simulink model "R2026b_pv_inverter_L_LC"  (R2026b)
settings: Solver=ode23tb  StopTime=0.3  MaxStep=2e-6  RelTol=1e-4  AbsTol=1e-6
libraries: ee_lib x13, nesl_utility x13, fl_lib x7
settings Model: Creator=35015  LastModifiedBy=35015
settings SimscapeCC: SimscapeLogType=all  SimscapeNominalValues="[{\"value\":\"1\",\"unit\":\"A\"},{\"value\":\"1\",\"unit\":\"bar\"},{\"value\":\"1\",\"unit\":\"cm^2\"},{\"value\":\"1\",\"unit\":\"cm^3/s\"},{\"value\":\"1\",\"unit\":\"kJ/kg\"},{\"value\":\"1\",\"unit\":\"kW\"},{\"value\":\"1\",\"unit\":\"l\"},{\"value\":\"1\",\"unit\":\"N\"},{\"value\":\"1\",\"unit\":\"N*m\"},{\"value\":\"1\",\"unit\":\"V\"},{\"value\":\"0.001\",\"unit\":\"Wb\"}]"  SimscapeUseEnergyAccounting=off

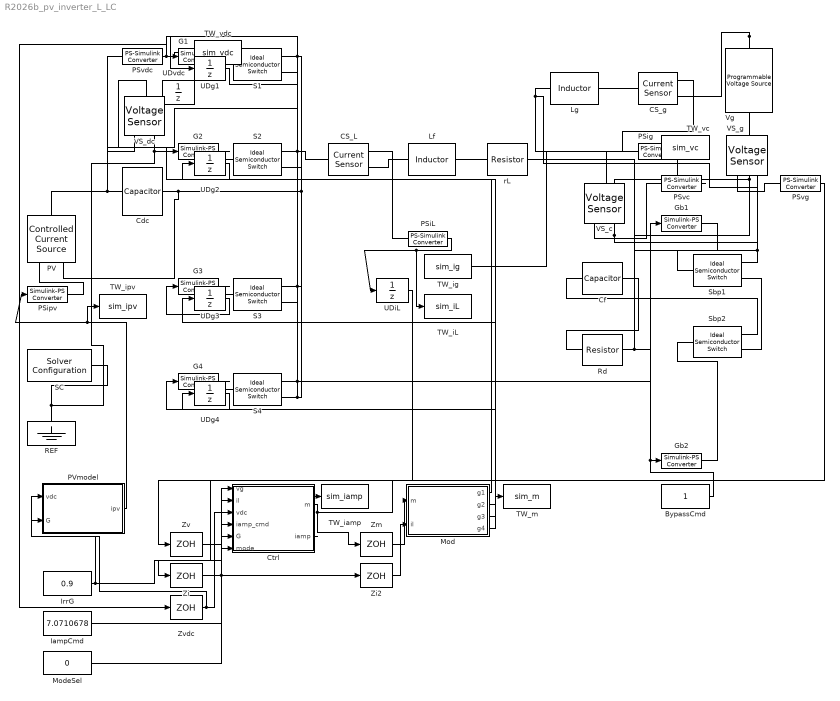
== system R2026b_pv_inverter_L_LC ==
  BypassCmd : Constant
  CS_L : fl_lib/Electrical/Electrical Sensors/Current Sensor
  CS_g : fl_lib/Electrical/Electrical Sensors/Current Sensor
  Cdc : ee_lib/Passive/Capacitor  cap_option=ee.enum.passive.capacitor.capOption.const  c=0.0045 F  Cvec=[1e-05, 1e-06] F  Vvec=[0, 10] V  CV_table_symmetry=ee.enum.passive.capacitor.tableSymmetry.yes  f_vec=[1, 10] kHz  DFext_vec=[.8, 1.2]  enable_C_tol=ee.enum.toleranceApplication.none  averaging_period=0 s  C_tol=5  tol_distribution=ee.enum.toleranceDistribution.uniform  nSigma=4  r=0 Ohm  g=0 1/Ohm  enable_operating_limits=ee.enum.enable.no  operating_limit_action=ee.enum.passive.reportOpLim.warn  max_working_voltage_range=[-25, 25] V  power_rating=1 W  maxTemperature=85 degC  thermalEnable=false  thermalMass=1 J/K  i_specify=off  i_priority=None  i=0 A  i_nominal_specify=off  i_nominal_value=1  i_nominal_unit=A  v_specify=off  v_priority=None  v=0 V  v_nominal_specify=off  v_nominal_value=1  v_nominal_unit=V  vc_specify=on  vc_priority=High  vc=75 V  vc_nominal_specify=off  vc_nominal_value=1  vc_nominal_unit=V  T_specify=off  T_priority=None  T=298.15 K  T_nominal_specify=off  T_nominal_value=1  T_nominal_unit=K
  Cf : ee_lib/Passive/Capacitor  cap_option=ee.enum.passive.capacitor.capOption.const  c=2e-05 F  Cvec=[1e-05, 1e-06] F  Vvec=[0, 10] V  CV_table_symmetry=ee.enum.passive.capacitor.tableSymmetry.yes  f_vec=[1, 10] kHz  DFext_vec=[.8, 1.2]  enable_C_tol=ee.enum.toleranceApplication.none  averaging_period=0 s  C_tol=5  tol_distribution=ee.enum.toleranceDistribution.uniform  nSigma=4  r=0 Ohm  g=0 1/Ohm  enable_operating_limits=ee.enum.enable.no  operating_limit_action=ee.enum.passive.reportOpLim.warn  max_working_voltage_range=[-25, 25] V  power_rating=1 W  maxTemperature=85 degC  thermalEnable=false  thermalMass=1 J/K  i_specify=off  i_priority=None  i=0 A  i_nominal_specify=off  i_nominal_value=1  i_nominal_unit=A  v_specify=off  v_priority=None  v=0 V  v_nominal_specify=off  v_nominal_value=1  v_nominal_unit=V  vc_specify=off  vc_priority=High  vc=0 V  vc_nominal_specify=off  vc_nominal_value=1  vc_nominal_unit=V  T_specify=off  T_priority=None  T=298.15 K  T_nominal_specify=off  T_nominal_value=1  T_nominal_unit=K
  Ctrl : MATLAB Function  TreatAsAtomicUnit=on
  G{1..4} (4 alike) : nesl_utility/Simulink-PS Converter  PhysicalDomain=network_engine_domain  SubClassName=ps_input  LeftPortType=input  RightPortType=output  PseudoPeriodic=off  Frequencies=[]  NoiseDistribution=none  NoiseParameters=[]  Unit=V  AffineConversion=off  FilteringAndDerivatives=provide  SimscapeFilterOrder=1  InputFilterTimeConstant=0.001  UdotUserProvided=0
  Gb1 : nesl_utility/Simulink-PS Converter  PhysicalDomain=network_engine_domain  SubClassName=ps_input  LeftPortType=input  RightPortType=output  PseudoPeriodic=off  Frequencies=[]  NoiseDistribution=none  NoiseParameters=[]  Unit=V  AffineConversion=off  FilteringAndDerivatives=provide  SimscapeFilterOrder=1  InputFilterTimeConstant=0.001  UdotUserProvided=0
  Gb2 : nesl_utility/Simulink-PS Converter  PhysicalDomain=network_engine_domain  SubClassName=ps_input  LeftPortType=input  RightPortType=output  PseudoPeriodic=off  Frequencies=[]  NoiseDistribution=none  NoiseParameters=[]  Unit=V  AffineConversion=off  FilteringAndDerivatives=provide  SimscapeFilterOrder=1  InputFilterTimeConstant=0.001  UdotUserProvided=0
  IampCmd : Constant  Value=7.0710678
  IrrG : Constant  Value=0.9
  Lf : ee_lib/Passive/Inductor  l=0.0005 H  enable_L_tol=ee.enum.toleranceApplication.none  L_tol=20  tol_distribution=ee.enum.toleranceDistribution.uniform  nSigma=4  r=0 Ohm  g=1e-9 1/Ohm  enable_operating_limits=ee.enum.enable.no  operating_limit_action=ee.enum.passive.reportOpLim.warn  max_working_current=1 A  power_rating=1 W  i_L_specify=off  i_L_priority=High  i_L=0 A  i_L_nominal_specify=off  i_L_nominal_value=1  i_L_nominal_unit=A
  Lg : ee_lib/Passive/Inductor  l=0.0005 H  enable_L_tol=ee.enum.toleranceApplication.none  L_tol=20  tol_distribution=ee.enum.toleranceDistribution.uniform  nSigma=4  r=0 Ohm  g=1e-9 1/Ohm  enable_operating_limits=ee.enum.enable.no  operating_limit_action=ee.enum.passive.reportOpLim.warn  max_working_current=1 A  power_rating=1 W  i_L_specify=off  i_L_priority=High  i_L=0 A  i_L_nominal_specify=off  i_L_nominal_value=1  i_L_nominal_unit=A
  Mod : MATLAB Function  TreatAsAtomicUnit=on
  ModeSel : Constant  Value=0
  PSiL : nesl_utility/PS-Simulink Converter  PhysicalDomain=network_engine_domain  SubClassName=ps_output  LeftPortType=input  RightPortType=output  PseudoPeriodic=off  Frequencies=[]  VectorFormat=inherit  Unit=A  AffineConversion=off
  PSig : nesl_utility/PS-Simulink Converter  PhysicalDomain=network_engine_domain  SubClassName=ps_output  LeftPortType=input  RightPortType=output  PseudoPeriodic=off  Frequencies=[]  VectorFormat=inherit  Unit=A  AffineConversion=off
  PSipv : nesl_utility/Simulink-PS Converter  PhysicalDomain=network_engine_domain  SubClassName=ps_input  LeftPortType=input  RightPortType=output  PseudoPeriodic=off  Frequencies=[]  NoiseDistribution=none  NoiseParameters=[]  Unit=A  AffineConversion=off  FilteringAndDerivatives=provide  SimscapeFilterOrder=1  InputFilterTimeConstant=0.001  UdotUserProvided=0
  PSvc : nesl_utility/PS-Simulink Converter  PhysicalDomain=network_engine_domain  SubClassName=ps_output  LeftPortType=input  RightPortType=output  PseudoPeriodic=off  Frequencies=[]  VectorFormat=inherit  Unit=V  AffineConversion=off
  PSvdc : nesl_utility/PS-Simulink Converter  PhysicalDomain=network_engine_domain  SubClassName=ps_output  LeftPortType=input  RightPortType=output  PseudoPeriodic=off  Frequencies=[]  VectorFormat=inherit  Unit=V  AffineConversion=off
  PSvg : nesl_utility/PS-Simulink Converter  PhysicalDomain=network_engine_domain  SubClassName=ps_output  LeftPortType=input  RightPortType=output  PseudoPeriodic=off  Frequencies=[]  VectorFormat=inherit  Unit=V  AffineConversion=off
  PV : fl_lib/Electrical/Electrical Sources/Controlled Current Source
  PVmodel : MATLAB Function  TreatAsAtomicUnit=on
  REF : fl_lib/Electrical/Electrical Elements/Electrical Reference
  Rd : ee_lib/Passive/Resistor  R=0.001 Ohm  enable_R_tol=ee.enum.toleranceApplication.none  R_tol=5  tol_distribution=ee.enum.toleranceDistribution.uniform  nSigma=4  enable_operating_limits=ee.enum.enable.no  operating_limit_action=ee.enum.passive.reportOpLim.warn  power_rating=1 W  max_working_voltage=100 V  noise_mode=ee.enum.sources.noise.Disabled  Tdevice=25 degC  sample_time=1e-3 s  repeatability=ee.enum.ic.repeatability.notRepeatable  user_seed=0  auto_seed=3890346746  power_derating_T1=70 degC  power_derating_T2=155 degC  operating_temperature_range_vec=[-50, 150] degC  alpha=3.93e-3 1/K  Tmeas=25 degC  thermal_mass=100 J/K  temperature_specify=off  temperature_priority=High  temperature=298.15 K  temperature_nominal_specify=off  temperature_nominal_value=1  temperature_nominal_unit=K
  S{1..4} (4 alike) : ee_lib/Semiconductors & Converters/Ideal Semiconductor Switch  port_option=ee.enum.controlport.ps  Ron=0.001 Ohm  Goff=1e-6 1/Ohm  Vth=0.5 V  diode_param=ee.enum.semiconductors.protectionDiode.nodynamics  diode_Vf=0.8 V  diode_Ron=0.001 Ohm  diode_Goff=1e-5 1/Ohm  diode_C=50e-9 F  diode_iRM=-235 A  diode_iF=300 A  diode_idot=-50 A/us  diode_trr_param=ee.enum.converters.diodetrr.trr_factor  diode_trr_factor=3  diode_trr=15 us  diode_Qrr=1500 s*uA
  SC : nesl_utility/Solver Configuration  PhysicalDomain=network_engine_domain  SubClassName=solver  LeftPortType=input  RightPortType=generic  Tones=[]  Harmonics=[]  SimulateNoise=off  Profile=off  UseLocalSampling=off  EnableSwitchedLinearOptims=on  FrequencyDomain=off  UseCCode=off  RelTol=0.001  AbsTol=0.001  MinStep=1e-09  ToWorkspace=off  RevertToSquareIcSolve=off  NumHomotopyIterations=100  PhasorMode=off  PhasorModeNumHarmonics=1  ConsistencySolver=NEWTON_XTOL_AFTER_FTOL  CanonicalOrdering=CANONICAL  OptimizeIntermediates=OPTIMIZED  MulticoreSolverChoice=BACKWARD_EULER  IndexReductionMethod=DerivativeReplacement  DoDC=off  ResidualTolerance=1e-09  ConsistencyTolSource=GLOBAL  ConsistencyAbsTol=0.001  ConsistencyRelTol=0.001  ConsistencyTolFactor=0.001  UseLocalSolver=off  LocalSolverChoice=NE_BACKWARD_EULER_ADVANCER  ResolveIndetEquations=on  FunctionEvalNumThread=1  LocalSolverSampleTime=0.001  DoFixedCost=off  MaxNonlinIter=3  MaxModeIter=2  ComputeImpulses=off  ImpulseIterations=2  LinearAlgebra=auto  LinearAlgebraNumThread=0  EquationFormulation=NE_TIME_EF  DelaysMemoryBudget=1024  AutomaticFiltering=on  FilteringTimeConstant=0.001  PartitionStorageMethod=AS_NEEDED  PartitionMemoryBudget=1024  PartitionMethod=BALANCED  MultibodyUseLocalSolver=off  MultibodyLocalSolverChoice=ODE1  MultibodyLocalSolverSampleTime=0.001
  Sbp1 : ee_lib/Semiconductors & Converters/Ideal Semiconductor Switch  port_option=ee.enum.controlport.ps  Ron=0.001 Ohm  Goff=1e-6 1/Ohm  Vth=0.5 V  diode_param=ee.enum.semiconductors.protectionDiode.nodynamics  diode_Vf=0.8 V  diode_Ron=0.001 Ohm  diode_Goff=1e-5 1/Ohm  diode_C=50e-9 F  diode_iRM=-235 A  diode_iF=300 A  diode_idot=-50 A/us  diode_trr_param=ee.enum.converters.diodetrr.trr_factor  diode_trr_factor=3  diode_trr=15 us  diode_Qrr=1500 s*uA
  Sbp2 : ee_lib/Semiconductors & Converters/Ideal Semiconductor Switch  port_option=ee.enum.controlport.ps  Ron=0.001 Ohm  Goff=1e-6 1/Ohm  Vth=0.5 V  diode_param=ee.enum.semiconductors.protectionDiode.nodynamics  diode_Vf=0.8 V  diode_Ron=0.001 Ohm  diode_Goff=1e-5 1/Ohm  diode_C=50e-9 F  diode_iRM=-235 A  diode_iF=300 A  diode_idot=-50 A/us  diode_trr_param=ee.enum.converters.diodetrr.trr_factor  diode_trr_factor=3  diode_trr=15 us  diode_Qrr=1500 s*uA
  TW_iL : ToWorkspace  VariableName=sim_iL  SaveFormat=Timeseries  SampleTime=2.5e-6
  TW_iamp : ToWorkspace  VariableName=sim_iamp  SaveFormat=Timeseries  SampleTime=5e-5
  TW_ig : ToWorkspace  VariableName=sim_ig  SaveFormat=Timeseries  SampleTime=2.5e-6
  TW_ipv : ToWorkspace  VariableName=sim_ipv  SaveFormat=Timeseries  SampleTime=2.5e-6
  TW_m : ToWorkspace  VariableName=sim_m  SaveFormat=Timeseries  SampleTime=5e-5
  TW_vc : ToWorkspace  VariableName=sim_vc  SaveFormat=Timeseries  SampleTime=2.5e-6
  TW_vdc : ToWorkspace  VariableName=sim_vdc  SaveFormat=Timeseries  SampleTime=2.5e-6
  UDg{1..4} (4 alike) : UnitDelay  SampleTime=2.5e-6
  UDiL : UnitDelay  SampleTime=2.5e-6
  UDvdc : UnitDelay  SampleTime=2.5e-6
  VS_c : fl_lib/Electrical/Electrical Sensors/Voltage Sensor
  VS_dc : fl_lib/Electrical/Electrical Sensors/Voltage Sensor
  VS_g : fl_lib/Electrical/Electrical Sensors/Voltage Sensor
  Vg : ee_lib/Sources/Programmable Voltage Source  magnitude_type=ee.enum.timechanging.constant  ac_magnitude=50.91168825 V  magn_ramp=1 V/s  magn_step=1 V  magn_modu_magn=1 V  magn_modu_freq=1 Hz  magn_t1=1 s  magn_t2=2 s  frequency_type=ee.enum.timechanging.constant  ac_frequency=50 Hz  freq_ramp=1 Hz/s  freq_step=1 Hz  freq_modu_magn=1 Hz  freq_modu_freq=1 Hz  freq_t1=1 s  freq_t2=2 s  phase_type=ee.enum.timechanging.constant  ac_shift=0 deg  phase_ramp=1 deg/s  phase_step=1 deg  phase_modu_magn=1 deg  phase_modu_freq=1 Hz  phase_t1=1 s  phase_t2=2 s  dc_type=ee.enum.timechanging.constant  dc_voltage=0 V  dc_ramp=1 V/s  dc_step=1 V  dc_modu_magn=1 V  dc_modu_freq=1 Hz  dc_t1=1 s  dc_t2=2 s  harmonic_option=0  harmonic_orders=[5, 7, 11, 13]  harmonic_ratios=[.1, .1, .1, .1]  harmonic_shifts=[0, 0, 0, 0] deg  harmonic_t1=-inf s  harmonic_t2=inf s  noise_mode=0  PSD=0 V^2/Hz  repeatability=1  auto_seed=0  user_seed=0  sample_time=1e-3 s  i_specify=off  i_priority=None  i=0 A  i_nominal_specify=off  i_nominal_value=1  i_nominal_unit=A  v_specify=off  v_priority=None  v=0 V  v_nominal_specify=off  v_nominal_value=1  v_nominal_unit=V
  Zi : ZeroOrderHold  SampleTime=5e-5
  Zi2 : ZeroOrderHold  SampleTime=2.5e-6
  Zm : ZeroOrderHold  SampleTime=2.5e-6
  Zv : ZeroOrderHold  SampleTime=5e-5
  Zvdc : ZeroOrderHold  SampleTime=5e-5
  rL : ee_lib/Passive/Resistor  R=0.1 Ohm  enable_R_tol=ee.enum.toleranceApplication.none  R_tol=5  tol_distribution=ee.enum.toleranceDistribution.uniform  nSigma=4  enable_operating_limits=ee.enum.enable.no  operating_limit_action=ee.enum.passive.reportOpLim.warn  power_rating=1 W  max_working_voltage=100 V  noise_mode=ee.enum.sources.noise.Disabled  Tdevice=25 degC  sample_time=1e-3 s  repeatability=ee.enum.ic.repeatability.notRepeatable  user_seed=0  auto_seed=3499211588  power_derating_T1=70 degC  power_derating_T2=155 degC  operating_temperature_range_vec=[-50, 150] degC  alpha=3.93e-3 1/K  Tmeas=25 degC  thermal_mass=100 J/K  temperature_specify=off  temperature_priority=High  temperature=298.15 K  temperature_nominal_specify=off  temperature_nominal_value=1  temperature_nominal_unit=K
  wires:
  PSvdc/1 -> Zvdc/1, TW_vdc/1
  PSvg/1 -> Zv/1
  PSiL/1 -> UDiL/1, TW_iL/1
  UDiL/1 -> Zi/1
  Zvdc/1 -> PVmodel/1(vdc), Ctrl/3(vdc)
  IrrG/1 -> PVmodel/2(G), Ctrl/5(G)
  PVmodel/1(ipv) -> PSipv/1, TW_ipv/1
  Zv/1 -> Ctrl/1(vg)
  Zi/1 -> Ctrl/2(il), Zi2/1
  IampCmd/1 -> Ctrl/4(iamp_cmd)
  ModeSel/1 -> Ctrl/6(mode)
  Ctrl/1(m) -> Zm/1, TW_m/1
  Zm/1 -> Mod/1(m)
  Zi2/1 -> Mod/2(il)
  Mod/1(g1) -> UDg1/1
  Mod/2(g2) -> UDg2/1
  Mod/3(g3) -> UDg3/1
  Mod/4(g4) -> UDg4/1
  UDg1/1 -> G1/1
  UDg2/1 -> G2/1
  UDg3/1 -> G3/1
  UDg4/1 -> G4/1
  BypassCmd/1 -> Gb1/1, Gb2/1
  PSig/1 -> TW_ig/1
  PSvc/1 -> TW_vc/1
  Ctrl/2(iamp) -> TW_iamp/1
  connections:
  PV/LConn1 -- Cdc/LConn1 -- S1/RConn1 -- S3/RConn1 -- VS_dc/LConn1
  PV/RConn2 -- Cdc/RConn1 -- S2/RConn2 -- S4/RConn2 -- VS_dc/RConn2 -- REF/LConn1 -- SC/RConn1
  S1/RConn2 -- S2/RConn1 -- CS_L/LConn1
  CS_L/RConn2 -- Lf/LConn1
  Lf/RConn1 -- rL/LConn1
  rL/RConn1 -- Sbp1/RConn1 -- Lg/LConn1 -- VS_c/LConn1
  Sbp1/RConn2 -- Sbp2/RConn2
  Sbp2/RConn1 -- Cf/LConn1
  Cf/RConn1 -- Rd/LConn1
  S3/RConn2 -- S4/RConn1 -- Rd/RConn1 -- Vg/RConn1 -- VS_c/RConn2 -- VS_g/RConn2
  Lg/RConn1 -- CS_g/LConn1
  Vg/LConn1 -- CS_g/RConn2 -- VS_g/LConn1
  CS_L/RConn1 -- PSiL/LConn1
  CS_g/RConn1 -- PSig/LConn1
  VS_dc/RConn1 -- PSvdc/LConn1
  VS_c/RConn1 -- PSvc/LConn1
  VS_g/RConn1 -- PSvg/LConn1
  PV/RConn1 -- PSipv/RConn1
  G1/RConn1 -- S1/LConn1
  G2/RConn1 -- S2/LConn1
  G3/RConn1 -- S3/LConn1
  G4/RConn1 -- S4/LConn1
  Gb1/RConn1 -- Sbp1/LConn1
  Gb2/RConn1 -- Sbp2/LConn1

== matlab function R2026b_pv_inverter_L_LC/Ctrl ==
  settings: updateMethod=DISCRETE  sampleTime=5e-5
  data: vg input; m output; il input; vdc input; iamp_cmd input; G input; mode input; iamp output
function [m, iamp] = ctrl(vg, il, vdc, iamp_cmd, G, mode)
%#codegen
% SOGI-PLL + 准PR(Tustin预畸变) + 电压环PI + P&O, 与 control_algos.py 同参数
Ts = 5e-5;
persistent th ia ib wq pii y1 y2 e1 e2 vint cnt pacc pn vref lastp dirp iampp init
if isempty(init)
    th = 0; ia = 0; ib = 0; wq = 2*pi*50; pii = 0;
    y1 = 0; y2 = 0; e1 = 0; e2 = 0; vint = 0;
    cnt = 0; pacc = 0; pn = 0; vref = 0.8*90; lastp = -1; dirp = 1; iampp = 0;
    init = 1;
end
w0 = 2*pi*50; ks = 1.41; kpp = 0.67; kip = 22; Um = 36*sqrt(2);
kppr = 4.7; kr = 300; wc = 5;
kpv = 0.2; kiv = 5; imin = 0; imax = 10;
dv = 0.5; vmin = 62; vmax = 75;
fsw = 20000; td = 4e-07; mlim = 0.95;
Iph = 2.9; I0 = 4.05e-8; nVT = 4.95;
kk = w0/tan(w0*Ts/2);
a0 = kk*kk + 2*wc*kk + w0*w0;
b0 = 2*kr*wc*kk/a0;
b2 = -2*kr*wc*kk/a0;
a1 = (-2*kk*kk + 2*w0*w0)/a0;
a2 = (kk*kk - 2*wc*kk + w0*w0)/a0;
% ---- SOGI-PLL ----
ia = ia + Ts*(ks*wq*(vg - ia) - wq*ib);
ib = ib + Ts*(wq*ia);
vq = ia*cos(th) + ib*sin(th);
vqn = vq/Um;
pii = pii + kip*vqn*Ts;
wq = w0 + kpp*vqn + pii;
th = th + wq*Ts;
if th > 2*pi
    th = th - 2*pi;
end
% ---- 电流幅值指令 ----
if mode < 0.5
    iampp = iamp_cmd;
else
    ipv = G*Iph - I0*(exp(vdc/nVT) - 1.0);
    pacc = pacc + vdc*ipv; pn = pn + 1;
    if mod(cnt, 20) == 0
        err = vdc - vref;
        o = kpv*err + vint;
        if ~((o >= imax && err > 0) || (o <= imin && err < 0))
            vint = vint + kiv*err*20*Ts;
        end
        iampp = kpv*err + vint;
        if iampp > imax, iampp = imax; end
        if iampp < imin, iampp = imin; end
    end
    if mod(cnt, 2000) == 0 && pn > 0
        pavg = pacc/pn;
        if lastp >= 0
            if pavg - lastp < 0
                dirp = -dirp;
            end
            vref = vref + dirp*dv;
            if vref > vmax, vref = vmax; end
            if vref < vmin, vref = vmin; end
        end
        lastp = pavg; pacc = 0; pn = 0;
    end
end
iamp = iampp;
% ---- 准PR 电流环 + 电网前馈 + 死区补偿 ----
iref = iamp*sin(th);
e = iref - il;
y = b0*e + b2*e2 - a1*y1 - a2*y2;
e2 = e1; e1 = e; y2 = y1; y1 = y;
u = kppr*e + y + vg;
u = u + 2*fsw*td*vdc*(1 - 2*(il < 0));
vdcs = vdc;
if vdcs < 10, vdcs = 10; end
lim = mlim*vdcs;
if u > lim, u = lim; end
if u < -lim, u = -lim; end
m = u/vdcs;
cnt = cnt + 1;
if cnt >= 2000
    cnt = 0;
end

== matlab function R2026b_pv_inverter_L_LC/PVmodel ==
  data: vdc input; ipv output; G input
function ipv = pv_current(vdc, G)
%#codegen
% 单二极管模型, 与 python/sim/pv_model.py 完全一致
Iph = 2.9; I0 = 4.05e-8; nVT = 4.95;
ipv = G*Iph - I0*(exp(vdc/nVT) - 1.0);

== matlab function R2026b_pv_inverter_L_LC/Mod ==
  settings: updateMethod=DISCRETE  sampleTime=2.5e-6
  data: m input; g1 output; il input; g2 output; g3 output; g4 output
function [g1, g2, g3, g4] = pwm(m, il)
%#codegen
% 单极性倍频 SPWM + 死区平均电压误差 (与 inverter_sim.py 同式)
persistent cnt
if isempty(cnt)
    cnt = 0;
end
fsw = 20000; td = 4e-07;
N = 20;
sgn = 1 - 2*(il < 0);
meff = m - 2*fsw*td*sgn;
if meff > 0.999, meff = 0.999; end
if meff < -0.999, meff = -0.999; end
carrier = 2*abs(cnt/N - 0.5);
duty = 0.5*(1 + meff);
sa = double(duty > carrier);
sb = double((1 - duty) > carrier);
g1 = sa; g2 = 1 - sa; g3 = sb; g4 = 1 - sb;
cnt = cnt + 1;
if cnt >= N
    cnt = 0;
end
